simulink model "SamplingModel_Abdulrahman"  (R2026a)
settings: Solver=VariableStepAuto  StopTime=20
libraries: dspxfrm3 x1, dspmlti4 x1, dspvision x1
settings Model: Creator=YazanK  LastModifiedBy=pc

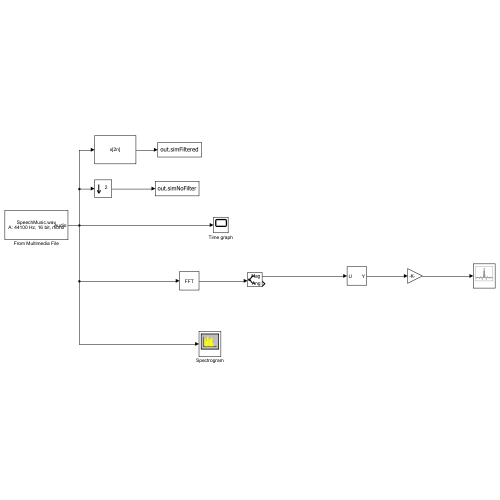
[thumbnail: Simulink's stored preview of the top-level diagram]
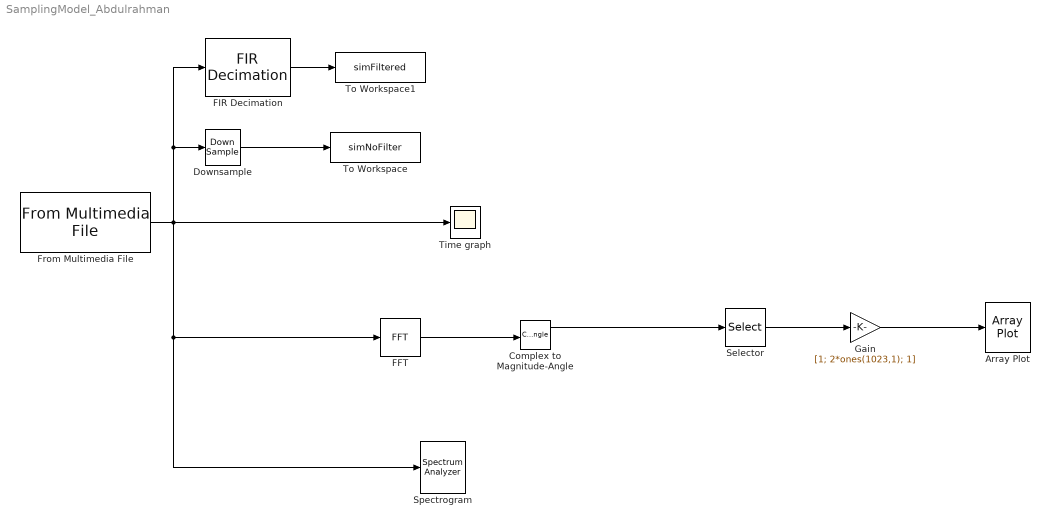
== system SamplingModel_Abdulrahman ==
  Array Plot : ArrayPlot  WindowPosition=[164.000000,123.000000,808.000000,611.000000,]  ScopeFrameLocation=window  SampleIncrement=21.533203125  MaximizeAxes=Off  YLimits=[-0.0026 0.023]
  Complex to Magnitude-Angle : ComplexToMagnitudeAngle
  Downsample : DownSample
  FFT : dspxfrm3/FFT  FFTImplementation=Auto  CompMethod=Table lookup  TableOpt=NEW  TableOptActive=Speed  BitRevOrder=off  Normalize=on  InheritFFTLength=on  FFTLength=64  WrapInput=on  roundingMode=Ceiling  overflowMode=off  firstCoeffDataTypeStr=Inherit: Same word length as input  firstCoeffLastDataTypeStr=Inherit: Same word length as input  outputMin=[]  outputMax=[]
  FIR Decimation : dspmlti4/FIR Decimation  FilterSource=Dialog parameters  h=filterCoefficients  D=2  filtStruct=Direct form  FilterObject=FDECIM  InputProcessing=Columns as channels (frame based)  framing=Enforce single-rate processing  AllowArbitraryInputLength=off  inputOffset=0  outputBufInitCond=0  roundingMode=Floor  overflowMode=off  firstCoeffDataTypeStr=Inherit: Same word length as input  firstCoeffMin=[]  firstCoeffMax=[]  firstCoeffLastDataTypeStr=Inherit: Same word length as input  outputDataTypeStr=Inherit: Same as accumulator  outputMin=[]  outputMax=[]  outputLastDataTypeStr=Inherit: Same as accumulator
  From Multimedia File : dspvision/From Multimedia File  inputFilename=Audios/SpeechMusic.wav  readRange=[1 Inf]  loop=on  numPlays=1  outputStreams=Audio only  videoDataType=single  audioDataType=double  inheritSampleTime=on  userDefinedSampleTime=1/30  noAudioOutput=off  isIntensityVideo=off  fourcc=RGB  colorVideoFormat=One multidimensional signal  outputEOF=off  dataOrg=Column-major  audioFrameSize=2048  computeAudioFrameSize=off  outSamplingMode=Sample based
      settings: LibrarySourceBlock=dspsrcs4/From Multimedia File
  Gain : Gain  Gain=[1; 2*ones(1023,1); 1]
  Selector : Selector  InputPortWidth=2048  IndexOptions=Index vector (dialog)  Indices=1:1025  OutputSizes=1
  Spectrogram : SpectrumAnalyzer  WindowPosition=[67.000000,-9.000000,958.000000,844.000000,]  ScopeFrameLocation=window  SpectrumType=Power density  ViewType=Spectrogram  Method=Welch  PlotAsTwoSidedSpectrum=off  FrequencyResolutionMethod=Window length  WindowInvariantSamplesPerUpdate=on  WindowLength=1323  FFTLengthSource=Property  FFTLength=2048  Span=22050  CenterFrequency=11025  StartFrequency=0  StopFrequency=22050  Window=Hamming  OverlapPercent=66.7  SpectrumUnits=dBW/Hz  TimeOrientation=Horizontal  TimeSpanSource=Property  TimeSpan=20  MaximizeAxes=Off  YLimits=[-120.8854793133496 7.496120686650402]  ColorLimits=[-132.87212 -41.4468]  AxesLayout=Horizontal  SelectedToolstripTab=spectrumAnalyzerToolstrip.estimationTab  DataDisplayPrecision=5
  Time graph : Scope
      settings: TimeUnits=Metric (based on Time Span)  ActiveDisplayYMinimum=-1.156982421875  ActiveDisplayYMaximum=1.21209716796875  YLabel=Amplitude
  To Workspace : ToWorkspace  VariableName=simNoFilter  SaveFormat=Timeseries  SampleTime=-1
  To Workspace1 : ToWorkspace  VariableName=simFiltered  SaveFormat=Timeseries  SampleTime=-1
  wires:
  From Multimedia File/1 -> FFT/1, Spectrogram/1, Time graph/1, Downsample/1, FIR Decimation/1
  FFT/1 -> Complex to Magnitude-Angle/1
  Complex to Magnitude-Angle/1 -> Selector/1
  Selector/1 -> Gain/1
  Gain/1 -> Array Plot/1
  Downsample/1 -> To Workspace/1
  FIR Decimation/1 -> To Workspace1/1
